simulink model "SixDegree"  (R2024b)
settings: Solver=ode4  StartTime=0.0  StopTime=150  FixedStep=0.001  RelTol=1e-3
PreLoadFcn:
  | run UnmannedAerialVehicle.m;
  | run aeroData_HGDGUO.m;
  | load op_trim3.mat
model workspace (MAT data in the model file):
  op_trim1 = opcond.OperatingReport
  op_trim1.TerminationString_ = '成功满足工作点设定。'
  op_trim1.OptimizationOutput_.iterations = 13
  op_trim1.OptimizationOutput_.funcCount = 248
  op_trim1.OptimizationOutput_.lssteplength = 1
  op_trim1.OptimizationOutput_.stepsize = 5.78862134999e-06
  op_trim1.OptimizationOutput_.algorithm = 'active-set'
  op_trim1.OptimizationOutput_.firstorderopt = 0
  op_trim1.OptimizationOutput_.constrviolation = 1.77591270585e-07
  op_trim1.OptimizationOutput_.message = '找到满足约束的局部最小值。
    | 
    | 优化已完成，因为目标函数沿
    | 可行方向在最优性容差值范围内呈现非递减，
    | 并且在约束容差值范围内满足约束。
    | 
    | <停止条件详细信息>
    | 
    | 优化已完成: 一阶最优性测度 0.000000e+00 小于
    | options.OptimalityTolerance = 1.000000e-06，并且最大约束违反值
    | 1.775913e-07 小于 options.ConstraintTolerance = 1.000000e-06。'
  op_trim1.OptimizationOutput_.bestfeasible.x = [41.0840297962; 0.294345069398; -0.740049530127; 7.79209597229e-12; -6.74692061789e-12; -500.06194579; 0.284965055514; -0.116413922122; 1.54482284055; -0.0752152769535; -0.0184984014468; -0.00578956736047; 0; -1.97416941445; 1.05553309513; 0.045613854234]
  op_trim1.OptimizationOutput_.bestfeasible.fval = 0
  op_trim1.OptimizationOutput_.bestfeasible.constrviolation = 1.77591270585e-07
  op_trim1.OptimizationOutput_.bestfeasible.firstorderopt = 0
  op_trim1.OptimizationOutput_.progress = {'<font face="monospaced"; size=3><BR>', '正在优化以求解所有所需的 dx/dt=0、x(k+1)-x(k)=0 和 y=ydes。<BR>', ' <BR>', '(最大误差)模块<BR>', ' ---------------------------------------------------------<BR>', '(3.52821e+00) SixDegree/u,v,w<BR>', '(3.51596e+00) SixDegree/u,v,w<BR>', '(3.48974e+00) SixDegree/u,v,w<BR>', '(3.36144e+00) SixDegree/p,q,r<BR>', '(8.49327e-01) SixDegree/p,q,r<BR>', '(1.05336e+00) SixDegree/u,v,w<BR>', '(9.99790e-01) SixDegree/u,v,w<BR>', '(1.08671e+00) SixDegree/u,v,w<BR>', '(1.12835e+00) SixDegree/u,v,w<BR>', '(6.01322e-01) SixDegree/u,v,w<BR>', '(8.89370e-02) SixDegree/u,v,w<BR>', '(2.04396e-03) SixDegree/u,v,w<BR>', '(1.77591e-07) SixDegree/xg,yg,zg<BR>', '(1.77591e-07) SixDegree/xg,yg,zg<BR>', ' <BR>', '成功满足工作点设定。<BR>'}
  op_trim1.Model_ = 'SixDegree'
  op_trim1.States_(1) = opcond.StateReport
  op_trim1.States_(1).dx_ = [0.204835866601; 2.01622528118e-08; -0.38315420244]
  op_trim1.States_(1).Nx_ = 3
  op_trim1.States_(1).Block_ = 'SixDegree/p,q,r'
  op_trim1.States_(1).x_ = [0.284965055514; -0.116413922122; 1.54482284055]
  op_trim1.States_(1).SteadyState_ = [0; 1; 0]
  op_trim1.States_(1).dxMin_ = [-Inf; -Inf; -Inf]
  op_trim1.States_(1).dxMax_ = [Inf; Inf; Inf]
  op_trim1.States_(1).Known_ = [0; 0; 0]
  op_trim1.States_(1).Min_ = [-Inf; -Inf; -Inf]
  op_trim1.States_(1).Max_ = [Inf; Inf; Inf]
  op_trim1.States_(2) = opcond.StateReport
  op_trim1.States_(2).dx_ = [0.256304007988; -3.04910683507e-08; 1.54946805891]
  op_trim1.States_(2).Nx_ = 3
  op_trim1.States_(2).Block_ = 'SixDegree/roll,pitch,yaw'
  op_trim1.States_(2).x_ = [-0.0752152769535; -0.0184984014468; -0.00578956736047]
  op_trim1.States_(2).SteadyState_ = [0; 1; 0]
  op_trim1.States_(2).dxMin_ = [-Inf; -Inf; -Inf]
  op_trim1.States_(2).dxMax_ = [Inf; Inf; Inf]
  op_trim1.States_(2).Known_ = [0; 0; 0]
  op_trim1.States_(2).Min_ = [-Inf; -Inf; -Inf]
  op_trim1.States_(2).Max_ = [Inf; Inf; Inf]
  op_trim1.States_(3) = opcond.StateReport
  op_trim1.States_(3).dx_ = [5.04275655544e-08; -64.5715205645; -6.46938436451e-09]
  op_trim1.States_(3).Nx_ = 3
  op_trim1.States_(3).Block_ = 'SixDegree/u,v,w'
  op_trim1.States_(3).x_ = [41.0840297962; 0.294345069398; -0.740049530127]
  op_trim1.States_(3).SteadyState_ = [1; 0; 1]
  op_trim1.States_(3).dxMin_ = [-Inf; -Inf; -Inf]
  op_trim1.States_(3).dxMax_ = [Inf; Inf; Inf]
  op_trim1.States_(3).Known_ = [0; 0; 0]
  op_trim1.States_(3).Min_ = [-Inf; -Inf; -Inf]
  op_trim1.States_(3).Max_ = [Inf; Inf; Inf]
  op_trim1.States_(4) = opcond.StateReport
  op_trim1.States_(4).dx_ = [41.0917487656; 1.77591270585e-07; 3.64908047112e-08]
  op_trim1.States_(4).Nx_ = 3
  op_trim1.States_(4).Block_ = 'SixDegree/xg,yg,zg'
  op_trim1.States_(4).x_ = [7.79209597229e-12; -6.74692061789e-12; -500.06194579]
  op_trim1.States_(4).SteadyState_ = [0; 1; 1]
  op_trim1.States_(4).dxMin_ = [-Inf; -Inf; -Inf]
  op_trim1.States_(4).dxMax_ = [Inf; Inf; Inf]
  op_trim1.States_(4).Known_ = [0; 0; 0]
  op_trim1.States_(4).Min_ = [-Inf; -Inf; -Inf]
  op_trim1.States_(4).Max_ = [Inf; Inf; Inf]
  op_trim1.Inputs_(1) = opcond.InputReport
  op_trim1.Inputs_(1).Block_ = 'SixDegree/delta T'
  op_trim1.Inputs_(1).PortWidth_ = 1
  op_trim1.Inputs_(1).PortDimensions_ = [1 1]
  op_trim1.Inputs_(1).Known_ = 0
  op_trim1.Inputs_(1).Min_ = -1
  op_trim1.Inputs_(1).Max_ = 1
  op_trim1.Inputs_(2) = opcond.InputReport
  op_trim1.Inputs_(2).Block_ = 'SixDegree/de'
  op_trim1.Inputs_(2).PortWidth_ = 1
  op_trim1.Inputs_(2).PortDimensions_ = [1 1]
  op_trim1.Inputs_(2).u_ = -1.97416941445
  op_trim1.Inputs_(2).Known_ = 0
  op_trim1.Inputs_(2).Min_ = -15
  op_trim1.Inputs_(2).Max_ = 15
  op_trim1.Inputs_(3) = opcond.InputReport
  op_trim1.Inputs_(3).Block_ = 'SixDegree/dr'
  op_trim1.Inputs_(3).PortWidth_ = 1
  op_trim1.Inputs_(3).PortDimensions_ = [1 1]
  op_trim1.Inputs_(3).u_ = 1.05553309513
  op_trim1.Inputs_(3).Known_ = 0
  op_trim1.Inputs_(3).Min_ = -15
  op_trim1.Inputs_(3).Max_ = 15
  op_trim1.Inputs_(4) = opcond.InputReport
  op_trim1.Inputs_(4).Block_ = 'SixDegree/da'
  op_trim1.Inputs_(4).PortWidth_ = 1
  op_trim1.Inputs_(4).PortDimensions_ = [1 1]
  op_trim1.Inputs_(4).u_ = 0.045613854234
  op_trim1.Inputs_(4).Known_ = 0
  op_trim1.Inputs_(4).Min_ = -15
  op_trim1.Inputs_(4).Max_ = 15
values from neighbouring files (symbols this model uses):
  aeroData = evalin('base','aeroData')    [CostTrim.m]    (also in aeroData_HGDGUO.mat = )
  b = evalin('base','b')    [CostTrim.m]    (also in UnmannedAerialVehicle.m = 10)
  cbar = evalin('base','cbar')    [CostTrim.m]    (also in UnmannedAerialVehicle.m = 1.32)
  CG = evalin('base','CG')    [CostTrim.m]    (also in UnmannedAerialVehicle.m = [0 0 0])
  CP = evalin('base','CP')    [CostTrim.m]    (also in UnmannedAerialVehicle.m = [3693.677 10.138 28.311]*1e-3)
  force_p1 = evalin('base','force_p1')    [CostTrim.m]    (also in UnmannedAerialVehicle.m = 2347)
  force_p2 = evalin('base','force_p2')    [CostTrim.m]    (also in UnmannedAerialVehicle.m = -32.38)
  I = [Ixx Ixy Ixz ... (first row only)    [UAVProperty.m]    (also in UnmannedAerialVehicle.m)
  Mass = evalin('base','Mass')    [CostTrim.m]    (also in UAVProperty.m = 600; UnmannedAerialVehicle.m = 600)
  S = evalin('base','S')    [CostTrim.m]    (also in UnmannedAerialVehicle.m = 13.2)
  torque_p1 = evalin('base','torque_p1')    [CostTrim.m]    (also in UnmannedAerialVehicle.m = 325.9)
  torque_p2 = evalin('base','torque_p2')    [CostTrim.m]    (also in UnmannedAerialVehicle.m = -5.774)
libraries: aerolibasang x2, simulink_extras x2, matrix_library x1, aerolibtransform2 x1, aerolibatmos2 x1
settings Model: Creator=LocoalKOH  LastModifiedBy=LocoalKOH
settings DataIOCC: ExternalInput=getinputstruct(op_trim3)  InitialState=getstatestruct(op_trim3)  LoadExternalInput=on  LoadInitialState=on

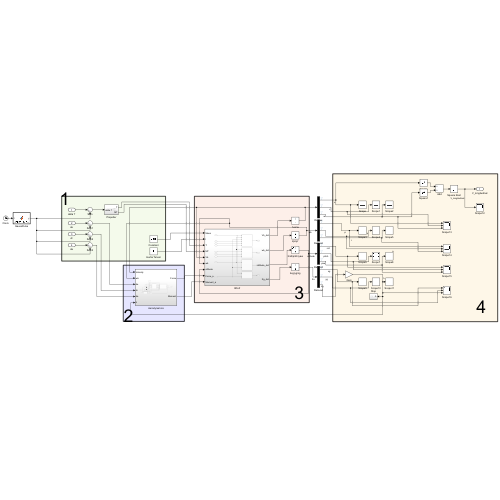
[thumbnail: Simulink's stored preview of the top-level diagram]
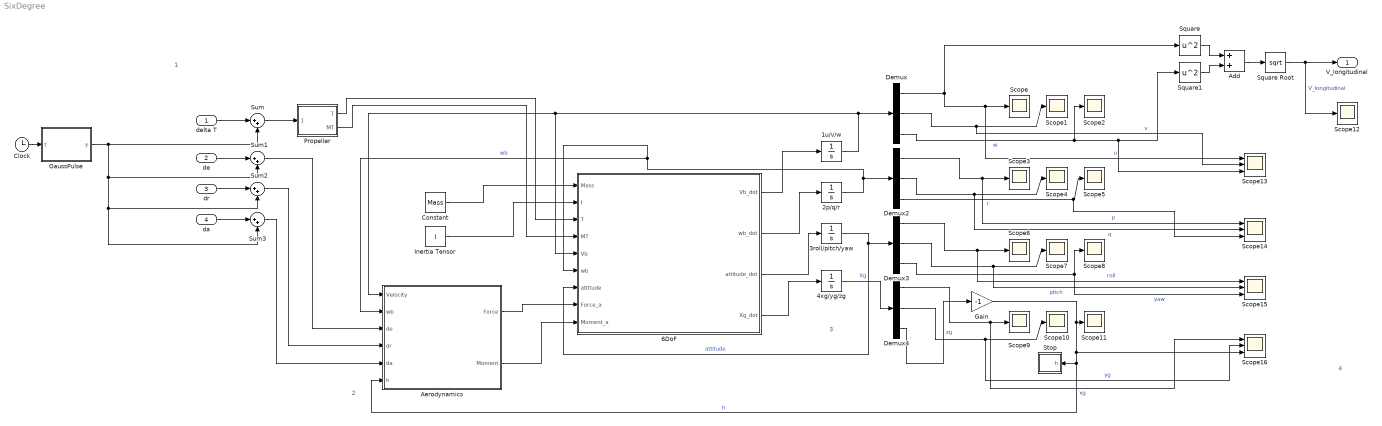
== system SixDegree ==
  note: 1
  note: 2
  note: 3
  note: 4
  delta T : Inport  OutDataTypeStr=double
  de : Inport  Port=2  OutDataTypeStr=double
  dr : Inport  Port=3  OutDataTypeStr=double
  da : Inport  Port=4  OutDataTypeStr=double
  1u/v/w : Integrator
  2p/q/r : Integrator
  3roll/pitch/yaw : Integrator  WrapState=on
  4xg/yg/zg : Integrator
  6DoF : Subsystem
  Add : Sum
  Aerodynamics : Subsystem
  Clock : Clock
  Constant : Constant  Value=Mass
  Demux{,2..4} (4 alike) : Demux  Outputs=3
  Gain : Gain  Gain=-1
  GaussPulse : MATLAB Function  TreatAsAtomicUnit=on
  Inertia Tensor : Constant  Value=I  VectorParams1D=off
  Propeller : Subsystem
  Scope{,1..12} (13 alike) : Scope
  Scope{13..16} (4 alike) : Scope  NumInputPorts=3
  Square : Math  Operator=square
  Square Root : Sqrt
  Square1 : Math  Operator=square
  Stop : Subsystem
  Sum{,1..3} (4 alike) : Sum  Inputs=|++
  V_longitudinal : Outport
  wires:
  Gain/1 -> Scope11/1, Scope16/3, Aerodynamics/6(h), Stop/1(h)  "h"
  2p/q/r/1 -> 6DoF/6(wb), Aerodynamics/2(wb), Demux2/1  "wb"
  3roll/pitch/yaw/1 -> 6DoF/7(attitude), Demux3/1  "attitude"
  4xg/yg/zg/1 -> Demux4/1  "Xg"
  1u/v/w/1 -> Aerodynamics/1(Velocity), 6DoF/5(Vb), Demux/1
  Demux/1 -> Scope13/1, Scope/1, Square/1  "u"
  Demux/2 -> Scope13/2, Scope1/1  "v"
  Demux/3 -> Scope2/1, Scope13/3, Square1/1  "w"
  Demux2/1 -> Scope14/1, Scope3/1  "p"
  Demux2/2 -> Scope14/2, Scope4/1  "q"
  Demux2/3 -> Scope14/3, Scope5/1  "r"
  Demux3/1 -> Scope15/1, Scope6/1  "roll"
  Demux3/2 -> Scope15/2, Scope7/1  "pitch"
  Demux3/3 -> Scope15/3, Scope8/1  "yaw"
  Demux4/1 -> Scope16/1, Scope9/1  "xg"
  Demux4/2 -> Scope16/2, Scope10/1  "yg"
  Constant/1 -> 6DoF/1(Mass)
  Inertia Tensor/1 -> 6DoF/2(I)
  6DoF/1(Vb_dot) -> 1u/v/w/1
  6DoF/2(wb_dot) -> 2p/q/r/1
  6DoF/3(attitude_dot) -> 3roll/pitch/yaw/1
  6DoF/4(Xg_dot) -> 4xg/yg/zg/1
  Demux4/3 -> Gain/1  "zg"
  Propeller/1(T) -> 6DoF/3(T)
  Propeller/2(MT) -> 6DoF/4(MT)
  Aerodynamics/1(Force) -> 6DoF/8(Force_a)
  Aerodynamics/2(Moment) -> 6DoF/9(Moment_a)
  Square/1 -> Add/1
  Square1/1 -> Add/2
  Add/1 -> Square Root/1
  Square Root/1 -> Scope12/1, V_longitudinal/1  "V_longitudinal"
  delta T/1 -> Sum/1
  Sum/1 -> Propeller/1(delta T)
  de/1 -> Sum1/1
  dr/1 -> Sum2/1
  da/1 -> Sum3/1
  Sum1/1 -> Aerodynamics/3(de)
  Sum2/1 -> Aerodynamics/4(dr)
  Sum3/1 -> Aerodynamics/5(da)
  GaussPulse/1(y) -> Sum3/2, Sum2/2, Sum1/2, Sum/2
  Clock/1 -> GaussPulse/1(t)

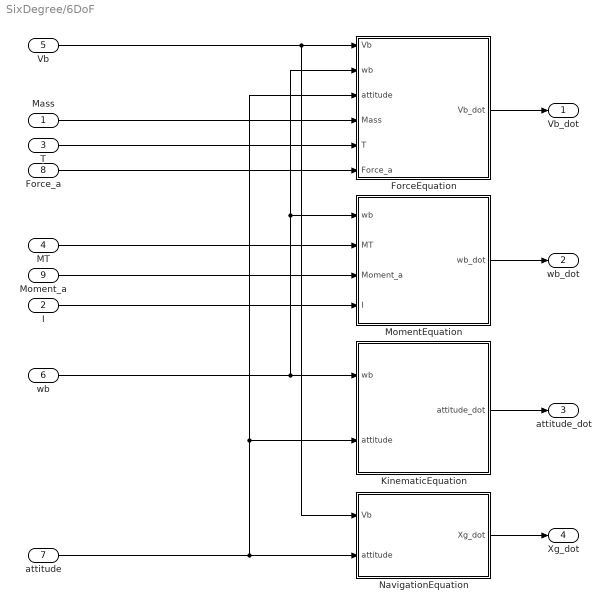
== system SixDegree/6DoF ==
  Mass : Inport
  I : Inport  Port=2
  T : Inport  Port=3
  MT : Inport  Port=4
  Vb : Inport  Port=5
  wb : Inport  Port=6
  attitude : Inport  Port=7
  Force_a : Inport  Port=8
  Moment_a : Inport  Port=9
  ForceEquation : MATLAB Function  TreatAsAtomicUnit=on
  KinematicEquation : MATLAB Function  TreatAsAtomicUnit=on
  MomentEquation : MATLAB Function  TreatAsAtomicUnit=on
  NavigationEquation : MATLAB Function  TreatAsAtomicUnit=on
  Vb_dot : Outport
  wb_dot : Outport  Port=2
  attitude_dot : Outport  Port=3
  Xg_dot : Outport  Port=4
  wires:
  wb/1 -> ForceEquation/2(wb), MomentEquation/1(wb), KinematicEquation/1(wb)
  NavigationEquation/1(Xg_dot) -> Xg_dot/1
  attitude/1 -> ForceEquation/3(attitude), KinematicEquation/2(attitude), NavigationEquation/2(attitude)
  T/1 -> ForceEquation/5(T)
  Moment_a/1 -> MomentEquation/3(Moment_a)
  KinematicEquation/1(attitude_dot) -> attitude_dot/1
  MT/1 -> MomentEquation/2(MT)
  I/1 -> MomentEquation/4(I)
  Force_a/1 -> ForceEquation/6(Force_a)
  MomentEquation/1(wb_dot) -> wb_dot/1
  ForceEquation/1(Vb_dot) -> Vb_dot/1
  Mass/1 -> ForceEquation/4(Mass)
  Vb/1 -> NavigationEquation/1(Vb), ForceEquation/1(Vb)

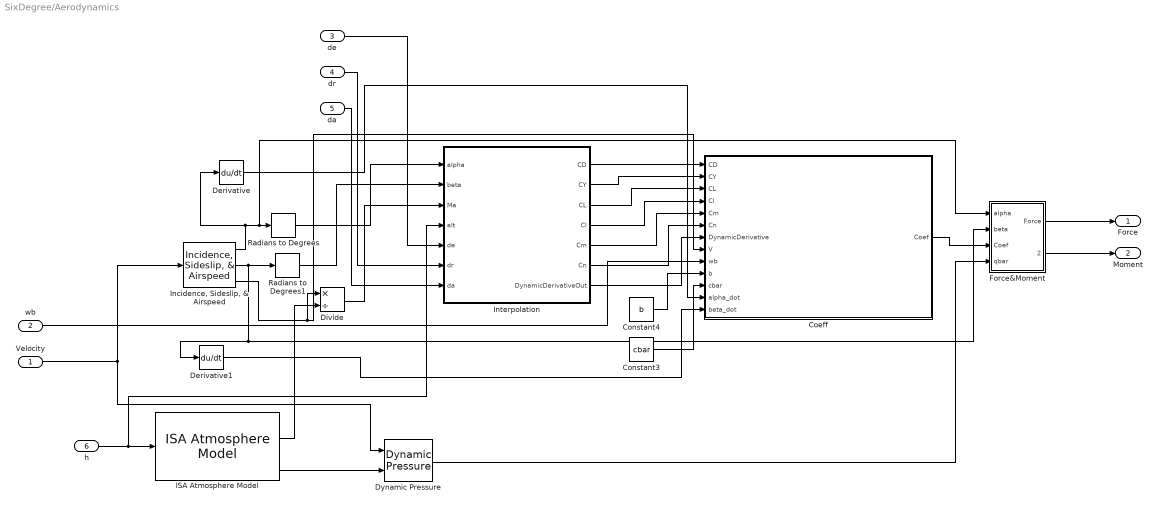
== system SixDegree/Aerodynamics ==
  Velocity : Inport
  wb : Inport  Port=2
  de : Inport  Port=3
  dr : Inport  Port=4
  da : Inport  Port=5
  h : Inport  Port=6
  Coeff : MATLAB Function  TreatAsAtomicUnit=on
  Constant3 : Constant  Value=cbar
  Constant4 : Constant  Value=b
  Derivative : Derivative
  Derivative1 : Derivative
  Divide : Product  Inputs=*/
  Dynamic Pressure : aerolibasang/Dynamic Pressure
  Force&Moment : Subsystem
  ISA Atmosphere Model : aerolibatmos2/ISA Atmosphere Model  useExtended=off  action=Warning  custom=off  viscosityOut=off  g=9.80665  gamma=1.4  R=287.0531  L=0.0065  h_trop=11000  h_strat=20000  rho0=1.225  P0=101325  T0=288.15  h0=0  S=110.4  Tref=273.15  muref=1.716e-5
  "Incidence, Sideslip, & Airspeed" : aerolibasang/Incidence, Sideslip, & Airspeed
  Interpolation : Subsystem
  Radians to Degrees : simulink_extras/Transformations/Radians to Degrees
  Radians to Degrees1 : simulink_extras/Transformations/Radians to Degrees
  Force : Outport
  Moment : Outport  Port=2
  wires:
  "Incidence, Sideslip, & Airspeed"/1 -> Derivative/1, Force&Moment/1(alpha), Radians to Degrees/1
  "Incidence, Sideslip, & Airspeed"/2 -> Force&Moment/2(beta), Derivative1/1, Radians to Degrees1/1
  h/1 -> Interpolation/4(alt), ISA Atmosphere Model/1
  ISA Atmosphere Model/4 -> Dynamic Pressure/2
  Dynamic Pressure/1 -> Force&Moment/4(qbar)
  Velocity/1 -> Dynamic Pressure/1, "Incidence, Sideslip, & Airspeed"/1
  Force&Moment/1(Force) -> Force/1
  Force&Moment/2(Moment) -> Moment/1
  Interpolation/1(CD) -> Coeff/1(CD)
  Interpolation/2(CY) -> Coeff/2(CY)
  Interpolation/3(CL) -> Coeff/3(CL)
  Interpolation/4(Cl) -> Coeff/4(Cl)
  Interpolation/5(Cm) -> Coeff/5(Cm)
  Interpolation/6(Cn) -> Coeff/6(Cn)
  Interpolation/7(DynamicDerivativeOut) -> Coeff/7(DynamicDerivative)
  Coeff/1(Coef) -> Force&Moment/3(Coef)
  Constant4/1 -> Coeff/10(b)
  Constant3/1 -> Coeff/11(cbar)
  Derivative/1 -> Coeff/12(alpha_dot)
  Derivative1/1 -> Coeff/13(beta_dot)
  "Incidence, Sideslip, & Airspeed"/3 -> Divide/1, Coeff/8(V)
  wb/1 -> Coeff/9(wb)
  Radians to Degrees/1 -> Interpolation/1(alpha)
  Radians to Degrees1/1 -> Interpolation/2(beta)
  de/1 -> Interpolation/5(de)
  dr/1 -> Interpolation/6(dr)
  da/1 -> Interpolation/7(da)
  Divide/1 -> Interpolation/3(Ma)
  ISA Atmosphere Model/2 -> Divide/2

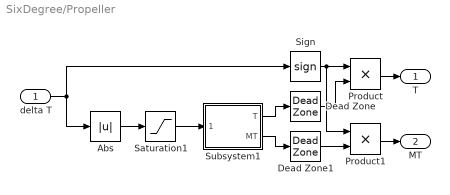
== system SixDegree/Propeller ==
  delta T : Inport
  Abs : Abs  SaturateOnIntegerOverflow=off
  Dead Zone : DeadZone  LowerValue=-Inf  UpperValue=0
  Dead Zone1 : DeadZone  LowerValue=-Inf  UpperValue=0
  Product : Product
  Product1 : Product
  Saturation1 : Saturate  UpperLimit=0.85  LowerLimit=0
  Sign : Signum
  Subsystem1 : Subsystem
  T : Outport
  MT : Outport  Port=2
  wires:
  Saturation1/1 -> Subsystem1/1(delta T)
  Subsystem1/2(MT) -> Dead Zone1/1
  delta T/1 -> Abs/1, Sign/1
  Dead Zone1/1 -> Product1/2
  Abs/1 -> Saturation1/1
  Dead Zone/1 -> Product/2
  Sign/1 -> Product1/1, Product/1
  Subsystem1/1(T) -> Dead Zone/1
  Product1/1 -> MT/1
  Product/1 -> T/1

== system SixDegree/Stop ==
  h : Inport
  One : Constant  OutDataTypeStr=Inherit: Inherit via back propagation
  Stop Simulation : Stop
  Switch : Switch  Criteria=u2 > Threshold  SaturateOnIntegerOverflow=off  InputSameDT=off
  Zero : Constant  Value=0  OutDataTypeStr=Inherit: Inherit via back propagation
  wires:
  One/1 -> Switch/3
  Zero/1 -> Switch/1
  Switch/1 -> Stop Simulation/1
  h/1 -> Switch/2

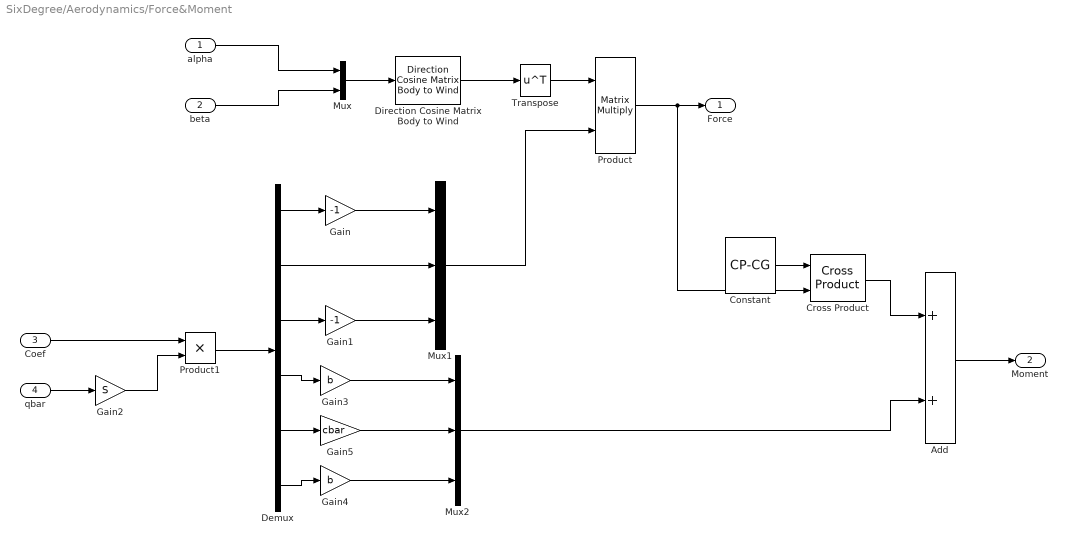
== system SixDegree/Aerodynamics/Force&Moment ==
  alpha : Inport
  beta : Inport  Port=2
  Coef : Inport  Port=3
  qbar : Inport  Port=4
  Add : Sum
  Constant : Constant  Value=CP-CG  VectorParams1D=off
  Cross Product : matrix_library/Cross Product
  Demux : Demux  Outputs=6
  Direction Cosine Matrix Body to Wind : aerolibtransform2/Direction Cosine Matrix Body to Wind
  Gain : Gain  Gain=-1
  Gain1 : Gain  Gain=-1
  Gain2 : Gain  Gain=S
  Gain3 : Gain  Gain=b
  Gain4 : Gain  Gain=b
  Gain5 : Gain  Gain=cbar
  Mux : Mux  Inputs=2
  Mux1 : Mux  Inputs=3
  Mux2 : Mux  Inputs=3
  Product : Product  Multiplication=Matrix(*)
  Product1 : Product
  Transpose : Math  Operator=transpose
  Force : Outport
  Moment : Outport  Port=2
  wires:
  Coef/1 -> Product1/1
  Gain/1 -> Mux1/1
  Demux/6 -> Gain4/1
  Demux/3 -> Gain1/1
  Product/1 -> Force/1, Cross Product/2
  Transpose/1 -> Product/1
  Gain4/1 -> Mux2/3
  Demux/4 -> Gain3/1
  Gain5/1 -> Mux2/2
  Direction Cosine Matrix Body to Wind/1 -> Transpose/1
  Product1/1 -> Demux/1
  Mux2/1 -> Add/2
  Demux/2 -> Mux1/2
  Mux1/1 -> Product/2
  Cross Product/1 -> Add/1
  Demux/5 -> Gain5/1
  Constant/1 -> Cross Product/1
  Add/1 -> Moment/1
  Gain3/1 -> Mux2/1
  Demux/1 -> Gain/1
  Gain2/1 -> Product1/2
  qbar/1 -> Gain2/1
  Gain1/1 -> Mux1/3
  Mux/1 -> Direction Cosine Matrix Body to Wind/1
  beta/1 -> Mux/2
  alpha/1 -> Mux/1

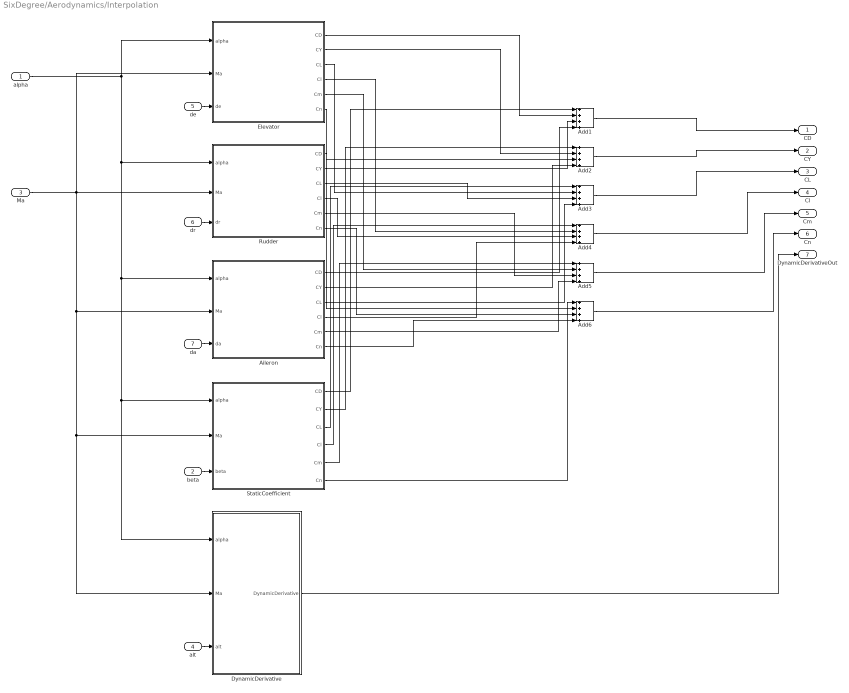
== system SixDegree/Aerodynamics/Interpolation ==
  alpha : Inport
  beta : Inport  Port=2
  Ma : Inport  Port=3
  alt : Inport  Port=4
  de : Inport  Port=5
  dr : Inport  Port=6
  da : Inport  Port=7
  Add{1..6} (6 alike) : Sum  Inputs=++++
  Aileron : Subsystem
  DynamicDerivative : Subsystem
  Elevator : Subsystem
  Rudder : Subsystem
  StaticCoefficient : Subsystem
  CD : Outport
  CY : Outport  Port=2
  CL : Outport  Port=3
  Cl : Outport  Port=4
  Cm : Outport  Port=5
  Cn : Outport  Port=6
  DynamicDerivativeOut : Outport  Port=7
  wires:
  StaticCoefficient/4(Cl) -> Add4/1
  StaticCoefficient/2(CY) -> Add2/1
  Add3/1 -> CL/1
  Aileron/3(CL) -> Add3/4
  Aileron/1(CD) -> Add1/4
  Rudder/4(Cl) -> Add4/3
  de/1 -> Elevator/3(de)
  StaticCoefficient/3(CL) -> Add3/1
  da/1 -> Aileron/3(da)
  Elevator/2(CY) -> Add2/2
  dr/1 -> Rudder/3(dr)
  StaticCoefficient/6(Cn) -> Add6/1
  alt/1 -> DynamicDerivative/3(alt)
  Aileron/6(Cn) -> Add6/4
  beta/1 -> StaticCoefficient/3(beta)
  Elevator/3(CL) -> Add3/2
  Aileron/4(Cl) -> Add4/4
  StaticCoefficient/1(CD) -> Add1/1
  Elevator/5(Cm) -> Add5/2
  Aileron/5(Cm) -> Add5/4
  Elevator/6(Cn) -> Add6/2
  Rudder/5(Cm) -> Add5/3
  Elevator/1(CD) -> Add1/2
  StaticCoefficient/5(Cm) -> Add5/1
  Rudder/1(CD) -> Add1/3
  Rudder/6(Cn) -> Add6/3
  Rudder/2(CY) -> Add2/3
  Aileron/2(CY) -> Add2/4
  Ma/1 -> DynamicDerivative/2(Ma), StaticCoefficient/2(Ma), Aileron/2(Ma), Rudder/2(Ma), Elevator/2(Ma)
  Add2/1 -> CY/1
  Rudder/3(CL) -> Add3/3
  Elevator/4(Cl) -> Add4/2
  DynamicDerivative/1(DynamicDerivative) -> DynamicDerivativeOut/1
  Add4/1 -> Cl/1
  Add6/1 -> Cn/1
  Add1/1 -> CD/1
  Add5/1 -> Cm/1
  alpha/1 -> DynamicDerivative/1(alpha), StaticCoefficient/1(alpha), Aileron/1(alpha), Rudder/1(alpha), Elevator/1(alpha)

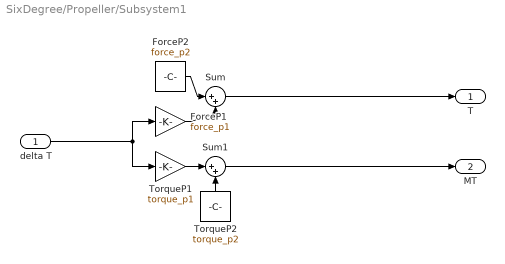
== system SixDegree/Propeller/Subsystem1 ==
  delta T : Inport
  ForceP1 : Gain  Gain=force_p1
  ForceP2 : Constant  Value=force_p2
  Sum : Sum  Inputs=|++
  Sum1 : Sum  Inputs=|++
  TorqueP1 : Gain  Gain=torque_p1
  TorqueP2 : Constant  Value=torque_p2
  T : Outport
  MT : Outport  Port=2
  wires:
  Sum/1 -> T/1
  delta T/1 -> TorqueP1/1, ForceP1/1
  ForceP1/1 -> Sum/2
  Sum1/1 -> MT/1
  TorqueP1/1 -> Sum1/1
  ForceP2/1 -> Sum/1
  TorqueP2/1 -> Sum1/2

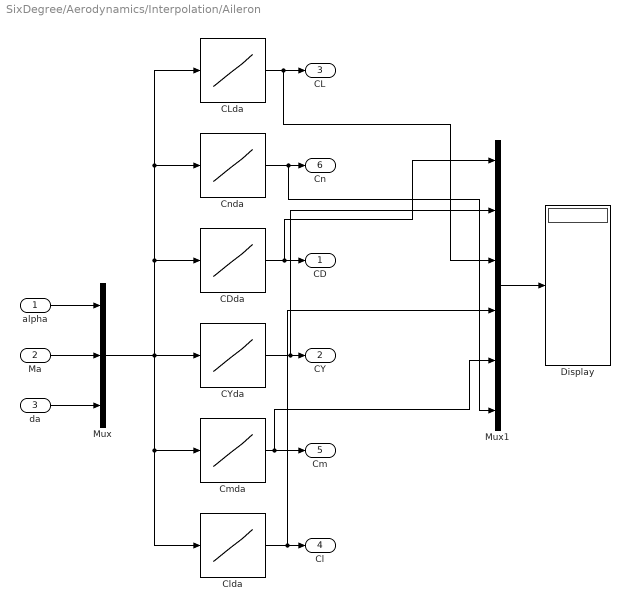
== system SixDegree/Aerodynamics/Interpolation/Aileron ==
  alpha : Inport
  Ma : Inport  Port=2
  da : Inport  Port=3
  CDda : Lookup_n-D  NumberOfTableDimensions=3  LookupTableObject=test  BreakpointsForDimension1=aeroData.Vec_alpha  BreakpointsForDimension2=aeroData.Vec_Ma  BreakpointsForDimension3=[-15 0 15]  UseOneInputPortForAllInputData=on  Table=aeroData.CD_alpha_Ma_da  InternalRulePriority=Speed  RndMeth=Simplest
  CLda : Lookup_n-D  NumberOfTableDimensions=3  LookupTableObject=test  BreakpointsForDimension1=aeroData.Vec_alpha  BreakpointsForDimension2=aeroData.Vec_Ma  BreakpointsForDimension3=[-15 0 15]  UseOneInputPortForAllInputData=on  Table=aeroData.CL_alpha_Ma_da  InternalRulePriority=Speed  RndMeth=Simplest
  CYda : Lookup_n-D  NumberOfTableDimensions=3  LookupTableObject=test  BreakpointsForDimension1=aeroData.Vec_alpha  BreakpointsForDimension2=aeroData.Vec_Ma  BreakpointsForDimension3=[-15 0 15]  UseOneInputPortForAllInputData=on  Table=aeroData.CY_alpha_Ma_da  InternalRulePriority=Speed  RndMeth=Simplest
  Clda : Lookup_n-D  NumberOfTableDimensions=3  LookupTableObject=test  BreakpointsForDimension1=aeroData.Vec_alpha  BreakpointsForDimension2=aeroData.Vec_Ma  BreakpointsForDimension3=[-15 0 15]  UseOneInputPortForAllInputData=on  Table=aeroData.Cl_alpha_Ma_da  InternalRulePriority=Speed  RndMeth=Simplest
  Cmda : Lookup_n-D  NumberOfTableDimensions=3  LookupTableObject=test  BreakpointsForDimension1=aeroData.Vec_alpha  BreakpointsForDimension2=aeroData.Vec_Ma  BreakpointsForDimension3=[-15 0 15]  UseOneInputPortForAllInputData=on  Table=aeroData.Cm_alpha_Ma_da  InternalRulePriority=Speed  RndMeth=Simplest
  Cnda : Lookup_n-D  NumberOfTableDimensions=3  LookupTableObject=test  BreakpointsForDimension1=aeroData.Vec_alpha  BreakpointsForDimension2=aeroData.Vec_Ma  BreakpointsForDimension3=[-15 0 15]  UseOneInputPortForAllInputData=on  Table=aeroData.Cn_alpha_Ma_da  InternalRulePriority=Speed  RndMeth=Simplest
  Display : Display
  Mux : Mux  Inputs=3
  Mux1 : Mux  Inputs=6
  CD : Outport
  CY : Outport  Port=2
  CL : Outport  Port=3
  Cl : Outport  Port=4
  Cm : Outport  Port=5
  Cn : Outport  Port=6
  wires:
  alpha/1 -> Mux/1
  Cnda/1 -> Mux1/6, Cn/1
  Ma/1 -> Mux/2
  da/1 -> Mux/3
  Mux/1 -> CYda/1, Cmda/1, Clda/1, Cnda/1, CLda/1, CDda/1
  CDda/1 -> Mux1/1, CD/1
  CLda/1 -> Mux1/3, CL/1
  CYda/1 -> Mux1/2, CY/1
  Cmda/1 -> Mux1/5, Cm/1
  Clda/1 -> Mux1/4, Cl/1
  Mux1/1 -> Display/1

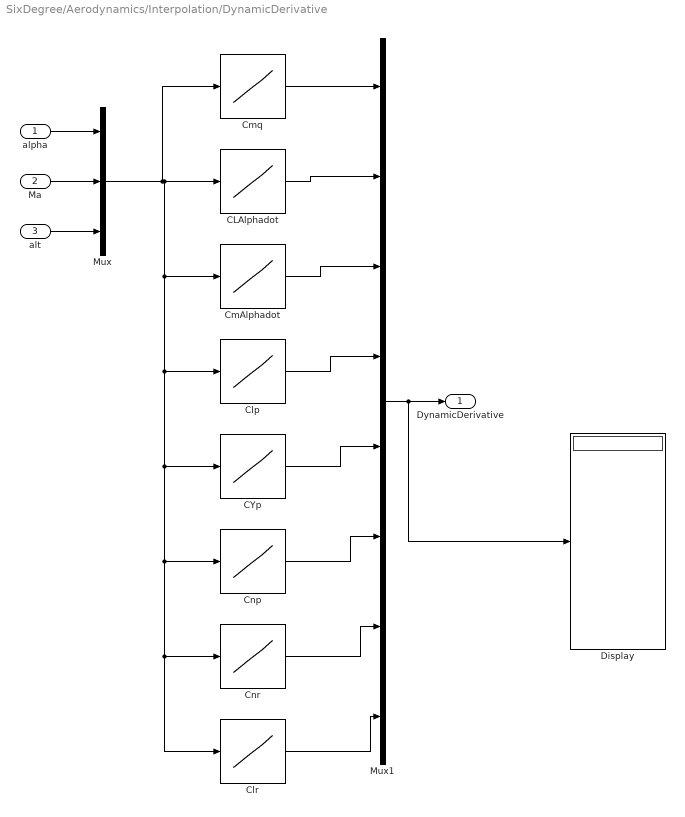
== system SixDegree/Aerodynamics/Interpolation/DynamicDerivative ==
  alpha : Inport
  Ma : Inport  Port=2
  alt : Inport  Port=3
  CLAlphadot : Lookup_n-D  NumberOfTableDimensions=3  LookupTableObject=test  BreakpointsForDimension1=aeroData.Vec_alpha2  BreakpointsForDimension2=aeroData.Vec_Ma2  BreakpointsForDimension3=aeroData.Vec_alt  UseOneInputPortForAllInputData=on  Table=aeroData.CLAlphadot_alpha_Ma_alt  InternalRulePriority=Speed  RndMeth=Simplest
  CYp : Lookup_n-D  NumberOfTableDimensions=3  LookupTableObject=test  BreakpointsForDimension1=aeroData.Vec_alpha2  BreakpointsForDimension2=aeroData.Vec_Ma2  BreakpointsForDimension3=aeroData.Vec_alt  UseOneInputPortForAllInputData=on  Table=aeroData.CYp_alpha_Ma_alt  InternalRulePriority=Speed  RndMeth=Simplest
  Clp : Lookup_n-D  NumberOfTableDimensions=3  LookupTableObject=test  BreakpointsForDimension1=aeroData.Vec_alpha2  BreakpointsForDimension2=aeroData.Vec_Ma2  BreakpointsForDimension3=aeroData.Vec_alt  UseOneInputPortForAllInputData=on  Table=aeroData.Clp_alpha_Ma_alt  InternalRulePriority=Speed  RndMeth=Simplest
  Clr : Lookup_n-D  NumberOfTableDimensions=3  LookupTableObject=test  BreakpointsForDimension1=aeroData.Vec_alpha2  BreakpointsForDimension2=aeroData.Vec_Ma2  BreakpointsForDimension3=aeroData.Vec_alt  UseOneInputPortForAllInputData=on  Table=aeroData.Clr_alpha_Ma_alt  InternalRulePriority=Speed  RndMeth=Simplest
  CmAlphadot : Lookup_n-D  NumberOfTableDimensions=3  LookupTableObject=test  BreakpointsForDimension1=aeroData.Vec_alpha2  BreakpointsForDimension2=aeroData.Vec_Ma2  BreakpointsForDimension3=aeroData.Vec_alt  UseOneInputPortForAllInputData=on  Table=aeroData.CmAlphadot_alpha_Ma_alt  InternalRulePriority=Speed  RndMeth=Simplest
  Cmq : Lookup_n-D  NumberOfTableDimensions=3  LookupTableObject=test  BreakpointsForDimension1=aeroData.Vec_alpha2  BreakpointsForDimension2=aeroData.Vec_Ma2  BreakpointsForDimension3=aeroData.Vec_alt  UseOneInputPortForAllInputData=on  Table=aeroData.Cmq_alpha_Ma_alt  InternalRulePriority=Speed  RndMeth=Simplest
  Cnp : Lookup_n-D  NumberOfTableDimensions=3  LookupTableObject=test  BreakpointsForDimension1=aeroData.Vec_alpha2  BreakpointsForDimension2=aeroData.Vec_Ma2  BreakpointsForDimension3=aeroData.Vec_alt  UseOneInputPortForAllInputData=on  Table=aeroData.Cnp_alpha_Ma_alt  InternalRulePriority=Speed  RndMeth=Simplest
  Cnr : Lookup_n-D  NumberOfTableDimensions=3  LookupTableObject=test  BreakpointsForDimension1=aeroData.Vec_alpha2  BreakpointsForDimension2=aeroData.Vec_Ma2  BreakpointsForDimension3=aeroData.Vec_alt  UseOneInputPortForAllInputData=on  Table=aeroData.Cnr_alpha_Ma_alt  InternalRulePriority=Speed  RndMeth=Simplest
  Display : Display
  Mux : Mux  Inputs=3
  Mux1 : Mux  Inputs=8
  DynamicDerivative : Outport
  wires:
  alpha/1 -> Mux/1
  Ma/1 -> Mux/2
  Clp/1 -> Mux1/4
  alt/1 -> Mux/3
  Mux/1 -> Clr/1, Cnr/1, Cnp/1, CYp/1, Clp/1, CmAlphadot/1, CLAlphadot/1, Cmq/1
  CLAlphadot/1 -> Mux1/2
  Cmq/1 -> Mux1/1
  CmAlphadot/1 -> Mux1/3
  CYp/1 -> Mux1/5
  Cnp/1 -> Mux1/6
  Cnr/1 -> Mux1/7
  Clr/1 -> Mux1/8
  Mux1/1 -> Display/1, DynamicDerivative/1

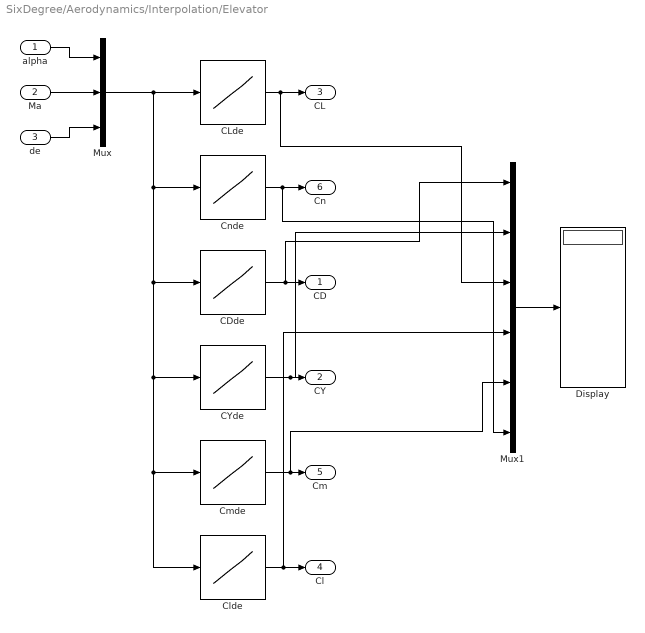
== system SixDegree/Aerodynamics/Interpolation/Elevator ==
  alpha : Inport
  Ma : Inport  Port=2
  de : Inport  Port=3
  CDde : Lookup_n-D  NumberOfTableDimensions=3  LookupTableObject=test  BreakpointsForDimension1=aeroData.Vec_alpha  BreakpointsForDimension2=aeroData.Vec_Ma  BreakpointsForDimension3=[-15 0 15]  UseOneInputPortForAllInputData=on  Table=aeroData.CD_alpha_Ma_de  InternalRulePriority=Speed  RndMeth=Simplest
  CLde : Lookup_n-D  NumberOfTableDimensions=3  LookupTableObject=test  BreakpointsForDimension1=aeroData.Vec_alpha  BreakpointsForDimension2=aeroData.Vec_Ma  BreakpointsForDimension3=[-15 0 15]  UseOneInputPortForAllInputData=on  Table=aeroData.CL_alpha_Ma_de  InternalRulePriority=Speed  RndMeth=Simplest
  CYde : Lookup_n-D  NumberOfTableDimensions=3  LookupTableObject=test  BreakpointsForDimension1=aeroData.Vec_alpha  BreakpointsForDimension2=aeroData.Vec_Ma  BreakpointsForDimension3=[-15 0 15]  UseOneInputPortForAllInputData=on  Table=aeroData.CY_alpha_Ma_de  InternalRulePriority=Speed  RndMeth=Simplest
  Clde : Lookup_n-D  NumberOfTableDimensions=3  LookupTableObject=test  BreakpointsForDimension1=aeroData.Vec_alpha  BreakpointsForDimension2=aeroData.Vec_Ma  BreakpointsForDimension3=[-15 0 15]  UseOneInputPortForAllInputData=on  Table=aeroData.Cl_alpha_Ma_de  InternalRulePriority=Speed  RndMeth=Simplest
  Cmde : Lookup_n-D  NumberOfTableDimensions=3  LookupTableObject=test  BreakpointsForDimension1=aeroData.Vec_alpha  BreakpointsForDimension2=aeroData.Vec_Ma  BreakpointsForDimension3=[-15 0 15]  UseOneInputPortForAllInputData=on  Table=aeroData.Cm_alpha_Ma_de  InternalRulePriority=Speed  RndMeth=Simplest
  Cnde : Lookup_n-D  NumberOfTableDimensions=3  LookupTableObject=test  BreakpointsForDimension1=aeroData.Vec_alpha  BreakpointsForDimension2=aeroData.Vec_Ma  BreakpointsForDimension3=[-15 0 15]  UseOneInputPortForAllInputData=on  Table=aeroData.Cn_alpha_Ma_de  InternalRulePriority=Speed  RndMeth=Simplest
  Display : Display
  Mux : Mux  Inputs=3
  Mux1 : Mux  Inputs=6
  CD : Outport
  CY : Outport  Port=2
  CL : Outport  Port=3
  Cl : Outport  Port=4
  Cm : Outport  Port=5
  Cn : Outport  Port=6
  wires:
  Cnde/1 -> Mux1/6, Cn/1
  alpha/1 -> Mux/1
  Mux/1 -> Clde/1, Cmde/1, CYde/1, CDde/1, Cnde/1, CLde/1
  Ma/1 -> Mux/2
  de/1 -> Mux/3
  CYde/1 -> Mux1/2, CY/1
  CDde/1 -> Mux1/1, CD/1
  CLde/1 -> Mux1/3, CL/1
  Cmde/1 -> Mux1/5, Cm/1
  Clde/1 -> Mux1/4, Cl/1
  Mux1/1 -> Display/1

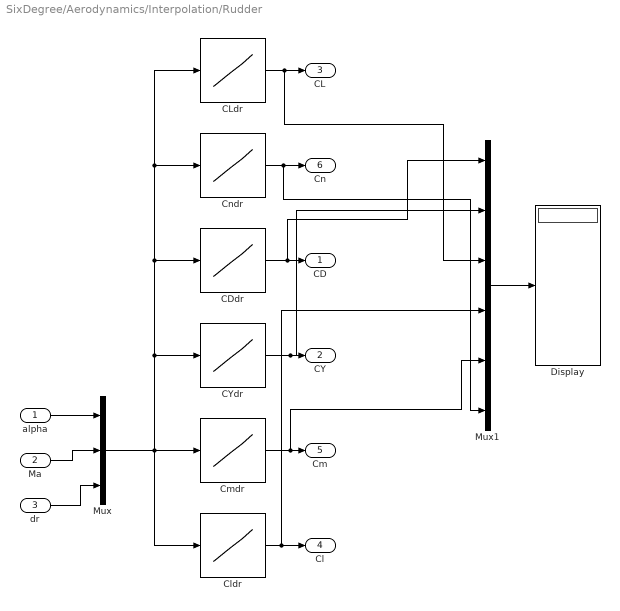
== system SixDegree/Aerodynamics/Interpolation/Rudder ==
  alpha : Inport
  Ma : Inport  Port=2
  dr : Inport  Port=3
  CDdr : Lookup_n-D  NumberOfTableDimensions=3  LookupTableObject=test  BreakpointsForDimension1=aeroData.Vec_alpha  BreakpointsForDimension2=aeroData.Vec_Ma  BreakpointsForDimension3=[-15 0 15]  UseOneInputPortForAllInputData=on  Table=aeroData.CD_alpha_Ma_dr  InternalRulePriority=Speed  RndMeth=Simplest
  CLdr : Lookup_n-D  NumberOfTableDimensions=3  LookupTableObject=test  BreakpointsForDimension1=aeroData.Vec_alpha  BreakpointsForDimension2=aeroData.Vec_Ma  BreakpointsForDimension3=[-15 0 15]  UseOneInputPortForAllInputData=on  Table=aeroData.CL_alpha_Ma_dr  InternalRulePriority=Speed  RndMeth=Simplest
  CYdr : Lookup_n-D  NumberOfTableDimensions=3  LookupTableObject=test  BreakpointsForDimension1=aeroData.Vec_alpha  BreakpointsForDimension2=aeroData.Vec_Ma  BreakpointsForDimension3=[-15 0 15]  UseOneInputPortForAllInputData=on  Table=aeroData.CY_alpha_Ma_dr  InternalRulePriority=Speed  RndMeth=Simplest
  Cldr : Lookup_n-D  NumberOfTableDimensions=3  LookupTableObject=test  BreakpointsForDimension1=aeroData.Vec_alpha  BreakpointsForDimension2=aeroData.Vec_Ma  BreakpointsForDimension3=[-15 0 15]  UseOneInputPortForAllInputData=on  Table=aeroData.Cl_alpha_Ma_dr  InternalRulePriority=Speed  RndMeth=Simplest
  Cmdr : Lookup_n-D  NumberOfTableDimensions=3  LookupTableObject=test  BreakpointsForDimension1=aeroData.Vec_alpha  BreakpointsForDimension2=aeroData.Vec_Ma  BreakpointsForDimension3=[-15 0 15]  UseOneInputPortForAllInputData=on  Table=aeroData.Cm_alpha_Ma_dr  InternalRulePriority=Speed  RndMeth=Simplest
  Cndr : Lookup_n-D  NumberOfTableDimensions=3  LookupTableObject=test  BreakpointsForDimension1=aeroData.Vec_alpha  BreakpointsForDimension2=aeroData.Vec_Ma  BreakpointsForDimension3=[-15 0 15]  UseOneInputPortForAllInputData=on  Table=aeroData.Cn_alpha_Ma_dr  InternalRulePriority=Speed  RndMeth=Simplest
  Display : Display
  Mux : Mux  Inputs=3
  Mux1 : Mux  Inputs=6
  CD : Outport
  CY : Outport  Port=2
  CL : Outport  Port=3
  Cl : Outport  Port=4
  Cm : Outport  Port=5
  Cn : Outport  Port=6
  wires:
  alpha/1 -> Mux/1
  CLdr/1 -> Mux1/3, CL/1
  Mux/1 -> Cmdr/1, Cldr/1, Cndr/1, CLdr/1, CDdr/1, CYdr/1
  Ma/1 -> Mux/2
  Cldr/1 -> Mux1/4, Cl/1
  dr/1 -> Mux/3
  Cndr/1 -> Mux1/6, Cn/1
  CDdr/1 -> Mux1/1, CD/1
  CYdr/1 -> Mux1/2, CY/1
  Cmdr/1 -> Mux1/5, Cm/1
  Mux1/1 -> Display/1

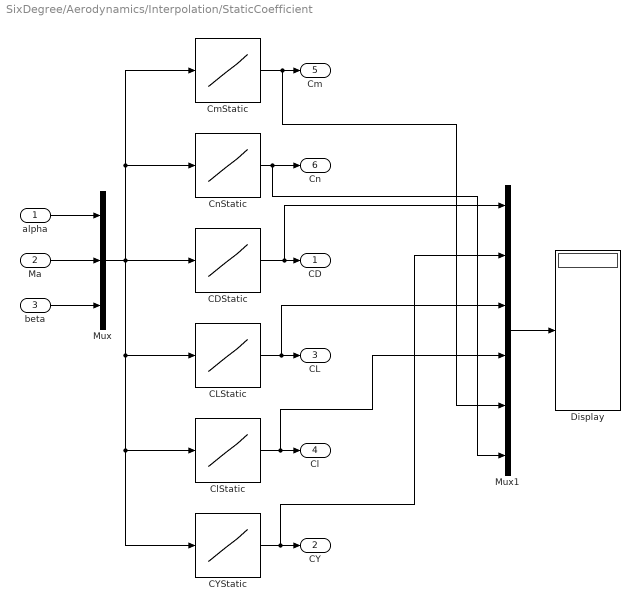
== system SixDegree/Aerodynamics/Interpolation/StaticCoefficient ==
  alpha : Inport
  Ma : Inport  Port=2
  beta : Inport  Port=3
  CDStatic : Lookup_n-D  NumberOfTableDimensions=3  LookupTableObject=test  BreakpointsForDimension1=aeroData.Vec_alpha  BreakpointsForDimension2=aeroData.Vec_Ma  BreakpointsForDimension3=aeroData.Vec_beta  UseOneInputPortForAllInputData=on  Table=aeroData.CD_alpha_Ma_beta  InternalRulePriority=Speed  RndMeth=Simplest
  CLStatic : Lookup_n-D  NumberOfTableDimensions=3  LookupTableObject=test  BreakpointsForDimension1=aeroData.Vec_alpha  BreakpointsForDimension2=aeroData.Vec_Ma  BreakpointsForDimension3=aeroData.Vec_beta  UseOneInputPortForAllInputData=on  Table=aeroData.CL_alpha_Ma_beta  InternalRulePriority=Speed  RndMeth=Simplest
  CYStatic : Lookup_n-D  NumberOfTableDimensions=3  LookupTableObject=test  BreakpointsForDimension1=aeroData.Vec_alpha  BreakpointsForDimension2=aeroData.Vec_Ma  BreakpointsForDimension3=aeroData.Vec_beta  UseOneInputPortForAllInputData=on  Table=aeroData.CY_alpha_Ma_beta  InternalRulePriority=Speed  RndMeth=Simplest
  ClStatic : Lookup_n-D  NumberOfTableDimensions=3  LookupTableObject=test  BreakpointsForDimension1=aeroData.Vec_alpha  BreakpointsForDimension2=aeroData.Vec_Ma  BreakpointsForDimension3=aeroData.Vec_beta  UseOneInputPortForAllInputData=on  Table=aeroData.Cl_alpha_Ma_beta  InternalRulePriority=Speed  RndMeth=Simplest
  CmStatic : Lookup_n-D  NumberOfTableDimensions=3  LookupTableObject=test  BreakpointsForDimension1=aeroData.Vec_alpha  BreakpointsForDimension2=aeroData.Vec_Ma  BreakpointsForDimension3=aeroData.Vec_beta  UseOneInputPortForAllInputData=on  Table=aeroData.Cm_alpha_Ma_beta  InternalRulePriority=Speed  RndMeth=Simplest
  CnStatic : Lookup_n-D  NumberOfTableDimensions=3  LookupTableObject=test  BreakpointsForDimension1=aeroData.Vec_alpha  BreakpointsForDimension2=aeroData.Vec_Ma  BreakpointsForDimension3=aeroData.Vec_beta  UseOneInputPortForAllInputData=on  Table=aeroData.Cn_alpha_Ma_beta  InternalRulePriority=Speed  RndMeth=Simplest
  Display : Display
  Mux : Mux  Inputs=3
  Mux1 : Mux  Inputs=6
  CD : Outport
  CY : Outport  Port=2
  CL : Outport  Port=3
  Cl : Outport  Port=4
  Cm : Outport  Port=5
  Cn : Outport  Port=6
  wires:
  alpha/1 -> Mux/1
  CmStatic/1 -> Mux1/5, Cm/1
  Mux/1 -> CYStatic/1, ClStatic/1, CLStatic/1, CmStatic/1, CnStatic/1, CDStatic/1
  Ma/1 -> Mux/2
  beta/1 -> Mux/3
  CLStatic/1 -> Mux1/3, CL/1
  CDStatic/1 -> Mux1/1, CD/1
  CnStatic/1 -> Mux1/6, Cn/1
  ClStatic/1 -> Mux1/4, Cl/1
  CYStatic/1 -> Mux1/2, CY/1
  Mux1/1 -> Display/1

== matlab function SixDegree/6DoF/KinematicEquation ==
  data: wb input; attitude_dot output size=[3 1]; attitude input
function attitude_dot = Kinematic(wb,attitude)
    p = wb(1);
    q = wb(2);
    r = wb(3);
    roll = attitude(1);
    pitch = attitude(2);
    A = [1,   sin(roll)*tan(pitch), cos(roll)*tan(pitch);
        0,   cos(roll),        -sin(roll);
        0,   sin(roll)/cos(pitch), cos(roll)/cos(pitch)];
    attitude_dot = A * [p; q; r];
end

== matlab function SixDegree/6DoF/MomentEquation ==
  data: wb input; MT input; Moment_a input; wb_dot output size=[3 1]; I input
function wb_dot = Moment(wb,MT,Moment_a,I)
    p = wb(1);
    q = wb(2);
    r = wb(3);
    Mx = Moment_a(1)+MT;
    My = Moment_a(2);
    Mz = Moment_a(3);
    Ixx = I(1,1);   Iyy = I(2,2);   Izz = I(3,3);
    Ixy = I(1,2);   Ixy = I(2,1);
    Iyz = I(2,3);   Iyz = I(3,2);
    Ixz = I(1,3);   Ixz = I(3,1);
    
    Sigma = - Izz*Ixy^2 + 2*Ixy*Ixz*Iyz - Iyy*Ixz^2 - Ixx*Iyz^2 + Ixx*Iyy*Izz;
    
    c1 = Iyy*Izz - Iyz^2;
    c2 = Ixz*Iyz - Ixy*Izz;
    c3 = Ixy*Iyz - Ixz*Iyy;
    c4 = Ixz^2*Iyz - Ixy^2*Iyz + Ixy*Ixz*Iyy - Ixy*Ixz*Izz;
    c5 = Ixy^2*Iyz - Ixz*Iyy*Ixy + Iyz^3 - Iyy*Izz*Iyz;
    c6 = - Ixz^2*Iyz + Ixy*Izz*Ixz - Iyz^3 + Iyy*Izz*Iyz;
    c7 = Ixz*Iyy^2 + 2*Ixz*Iyz^2 + Ixx*Ixy*Iyz - Ixx*Ixz*Iyy - Ixy*Iyy*Iyz - Ixy*Iyz*Izz - Ixz*Iyy*Izz;
    c8 = Ixy^2*Izz - Ixz^2*Iyy + Iyy^2*Izz - Iyy*Iyz^2 - Iyy*Izz^2 + Iyz^2*Izz;
    c9 = Ixx*Ixy*Izz - Ixy*Izz^2 - Ixx*Ixz*Iyz - 2*Ixy*Iyz^2 + Ixz*Iyy*Iyz + Ixy*Iyy*Izz + Ixz*Iyz*Izz;
    
    p_dot = ...
        (c1/Sigma)*Mx ...
        + (c2/Sigma)*My ...
        + (c3/Sigma)*Mz ...
        + (c4/Sigma)*p^2 ...
        + (c5/Sigma)*q^2 ...
        + (c6/Sigma)*r^2 ...
        + (c7/Sigma)*p*q ...
        + (c8/Sigma)*q*r ...
        + (c9/Sigma)*p*r;
    
    c10 = Ixz*Iyz - Ixy*Izz;
    c11 = Ixx*Izz - Ixz^2;
    c12 = Ixy*Ixz - Ixx*Iyz;
    c13 = - Ixy^2*Ixz + Ixx*Iyz*Ixy - Ixz^3 + Ixx*Izz*Ixz;
    c14 = Ixy^2*Ixz - Ixz*Iyz^2 - Ixx*Ixy*Iyz + Ixy*Iyz*Izz;
    c15 = Ixz^3 + Ixz*Iyz^2 - Ixx*Izz*Ixz - Ixy*Izz*Iyz;
    c16 = Ixx*Ixy*Ixz - 2*Ixz^2*Iyz - Ixx^2*Iyz - Ixy*Ixz*Iyy + Ixx*Iyy*Iyz + Ixy*Ixz*Izz + Ixx*Iyz*Izz;
    c17 = 2*Ixy*Ixz^2 + Ixy*Izz^2 - Ixx*Ixz*Iyz - Ixx*Ixy*Izz + Ixz*Iyy*Iyz - Ixy*Iyy*Izz - Ixz*Iyz*Izz;
    c18 = - Ixx^2*Izz + Ixx*Ixz^2 + Ixx*Iyz^2 + Ixx*Izz^2 - Ixy^2*Izz - Ixz^2*Izz;
    
    q_dot = ...
        (c10/Sigma)*Mx ...
        + (c11/Sigma)*My ...
        + (c12/Sigma)*Mz ...
        + (c13/Sigma)*p^2 ...
        + (c14/Sigma)*q^2 ...
        + (c15/Sigma)*r^2 ...
        + (c16/Sigma)*p*q ...
        + (c17/Sigma)*q*r ...
        + (c18/Sigma)*p*r;
    
    c19 = Ixy*Iyz - Ixz*Iyy;
    c20 = Ixy*Ixz - Ixx*Iyz;
    c21 = Ixx*Iyy - Ixy^2;
    c22 = Ixy^3 + Ixy*Ixz^2 - Ixx*Iyy*Ixy - Ixx*Iyz*Ixz;
    c23 = - Ixy^3 - Ixy*Iyz^2 + Ixx*Iyy*Ixy + Ixz*Iyy*Iyz;
    c24 = Ixy*Iyz^2 - Ixy*Ixz^2 + Ixx*Ixz*Iyz - Ixz*Iyy*Iyz;
    c25 = Ixx^2*Iyy - Ixx*Ixy^2 - Ixx*Iyy^2 - Ixx*Iyz^2 + Ixy^2*Iyy + Ixz^2*Iyy;
    c26 = Ixx*Ixy*Iyz - Ixz*Iyy^2 - 2*Ixy^2*Ixz + Ixx*Ixz*Iyy + Ixy*Iyy*Iyz - Ixy*Iyz*Izz + Ixz*Iyy*Izz;
    c27 = Ixx^2*Iyz + 2*Ixy^2*Iyz - Ixx*Ixy*Ixz - Ixy*Ixz*Iyy - Ixx*Iyy*Iyz + Ixy*Ixz*Izz - Ixx*Iyz*Izz;
    
    r_dot = ...
        (c19/Sigma)*Mx ...
        + (c20/Sigma)*My ...
        + (c21/Sigma)*Mz ...
        + (c22/Sigma)*p^2 ...
        + (c23/Sigma)*q^2 ...
        + (c24/Sigma)*r^2 ...
        + (c25/Sigma)*p*q ...
        + (c26/Sigma)*q*r ...
        + (c27/Sigma)*p*r;
    
    wb_dot = [p_dot;q_dot;r_dot];
end

== matlab function SixDegree/6DoF/NavigationEquation ==
  data: Vb input; Xg_dot output size=[3 1]; attitude input
function Xg_dot = Navigation(Vb,attitude)
    roll = attitude(1);
    pitch = attitude(2);
    yaw = attitude(3);
    CEB=[                cos(pitch)*cos(yaw),     cos(pitch)*sin(yaw),               -sin(pitch);
        sin(pitch)*cos(yaw)*sin(roll)-sin(yaw)*cos(roll),sin(pitch)*sin(yaw)*sin(roll)+cos(yaw)*cos(roll),cos(pitch)*sin(roll);
        sin(pitch)*cos(yaw)*cos(roll)+sin(yaw)*sin(roll),sin(pitch)*sin(yaw)*cos(roll)-cos(yaw)*sin(roll),cos(pitch)*cos(roll)];
    Xg_dot = CEB'*Vb;
end

== matlab function SixDegree/6DoF/ForceEquation ==
  data: Vb input; Vb_dot output size=[3 1]; wb input; attitude input; Mass input; T input; Force_a input
function Vb_dot = Force(Vb,wb,attitude,Mass,T,Force_a)
    u = Vb(1);
    v = Vb(2);
    w = Vb(3);
    p = wb(1);
    q = wb(2);
    r = wb(3);
    roll = attitude(1);
    pitch = attitude(2);
    %角速度、线速度耦合项
    fwv=Mass*[v*r-w*q;
        -u*r+w*p;
        u*q-v*p;];
    %重力
    g = 9.80665;
    G=Mass*[-g*sin(pitch);
        g*cos(pitch)*sin(roll);
        g*cos(pitch)*cos(roll)];
    %推力
    Force = [T;0;0];
    
    Vb_dot = (fwv+G+Force+Force_a)/Mass;
end

== matlab function SixDegree/GaussPulse ==
  data: t input; y output
function y = gauss_pulse(t)
    y = 0.1 * exp(-(t - 5)^2 / 0.1);  % 在t=5秒附近有扰动
end

== matlab function SixDegree/Aerodynamics/Coeff ==
  data: Coef output; CD input; CY input; CL input; Cl input; Cm input; Cn input; DynamicDerivative input; V input; wb input; b input; cbar input; alpha_dot input; beta_dot input
function Coef = CoefficientCalculator(CD,CY,CL,Cl,Cm,Cn,DynamicDerivative,V,wb,b,cbar,alpha_dot,beta_dot)
    p = wb(1);
    q = wb(2);
    r = wb(3);
    
    Cmq = DynamicDerivative(1);
    CLalphadot = DynamicDerivative(2);
    Cmalphadot = DynamicDerivative(3);
    Clp = DynamicDerivative(4);
    CYp = DynamicDerivative(5);
    Cnp = DynamicDerivative(6);
    Cnr = DynamicDerivative(7);
    Clr = DynamicDerivative(8);

    CD_dynamic = 0;
    CL_dynamic = CLalphadot*(alpha_dot*cbar/(2*V));
    CY_dynamic = CYp*(p*b/(2*V));
    Cl_dynamic = Clp*(p*b/(2*V)) + Clr*(r*b/(2*V));
    Cm_dynamic = Cmq*(q*cbar/(2*V)) + Cmalphadot*(alpha_dot*cbar/(2*V));
    Cn_dynamic = Cnp*(p*b/(2*V)) + Cnr*(r*b/(2*V));

    CD_sum = CD + CD_dynamic;
    CL_sum = CL + CL_dynamic;
    CY_sum = CY + CY_dynamic;
    Cl_sum = Cl + Cl_dynamic;
    Cm_sum = Cm + Cm_dynamic;
    Cn_sum = Cn + Cn_dynamic;

    Coef = [CD_sum; CY_sum; CL_sum; Cl_sum; Cm_sum; Cn_sum];
end
